simulink model "LCC_C"  (R2026b)
settings: Solver=ode23t  StopTime=5e-6
InitFcn:
  | % LCC-C WPT Inverse Design
  | % All values use SI units
  | 
  | %% 1. Known parameters
  | F = 13.56e6;       % Frequency (Hz)
  | V = 173.2;            % Peak voltage (V), P_in = 500w
  | 
  | L_1 = 486e-9;      % Transmitter coil (H)
  | L_2 = 486e-9; % Receiver coil (H)
  | L21 = 90e-9
  | 
  | R_l = 12.5;        % Load resistance (Ohm)
  | Z_in = 30;         % Target input impedance (Ohm)
  | 
  | Q_1 = 951.1;       % Transmitter quality factor
  | Q_2 = 931;         % Receiver quality factor
  | 
  | %% 2. Derived parameters
  | omega = 2*pi*F;
  | T = 1/F;
  | 
  | % Load quality factor
  | Q_load = omega*L_2/R_l;
  | 
  | % Coupling coefficient from optimal load condition
  | k = sqrt(((Q_2/Q_load)^2-1)/(Q_1*Q_2));
  | 
  | % Mutual inductance
  | M = k*sqrt(L_1*L_2);
  | 
  | % LCC compensation inductor
  | L = M*sqrt(Z_in/R_l);
  | 
  | % LCC parallel compensation capacitor
  | C = 1/(omega^2*L);
  | 
  | % Transmitter series capacitor
  | C_1 = 1/(omega^2*(L_1-L));
  | 
  | % Receiver series capacitor
  | C_2 = 1/(omega^2*(L_2+L21));
  | 
  | %% 3. Additional calculated quantities
  | R_1 = omega*L_1/Q_1;
  | R_2 = omega*L_2/Q_2;
  | 
  | Q_load_opt = Q_2/sqrt(1+k^2*Q_1*Q_2);
  | Z_in_check = (L/M)^2*R_l;
  | 
  | I_in_pk_ideal = V/Z_in;
  | P_in_ideal = V^2/(2*Z_in);
libraries: fl_lib x54, nesl_utility x33
settings Model: Creator=charl  LastModifiedBy=charl
settings SimscapeCC: SimscapeLogType=all  SimscapeNominalValues="[{\"value\":\"1\",\"unit\":\"A\"},{\"value\":\"1\",\"unit\":\"bar\"},{\"value\":\"1\",\"unit\":\"cm^2\"},{\"value\":\"1\",\"unit\":\"cm^3/s\"},{\"value\":\"1\",\"unit\":\"kJ/kg\"},{\"value\":\"1\",\"unit\":\"kW\"},{\"value\":\"1\",\"unit\":\"l\"},{\"value\":\"1\",\"unit\":\"N\"},{\"value\":\"1\",\"unit\":\"N*m\"},{\"value\":\"1\",\"unit\":\"V\"},{\"value\":\"0.001\",\"unit\":\"Wb\"}]"  SimscapeUseEnergyAccounting=off

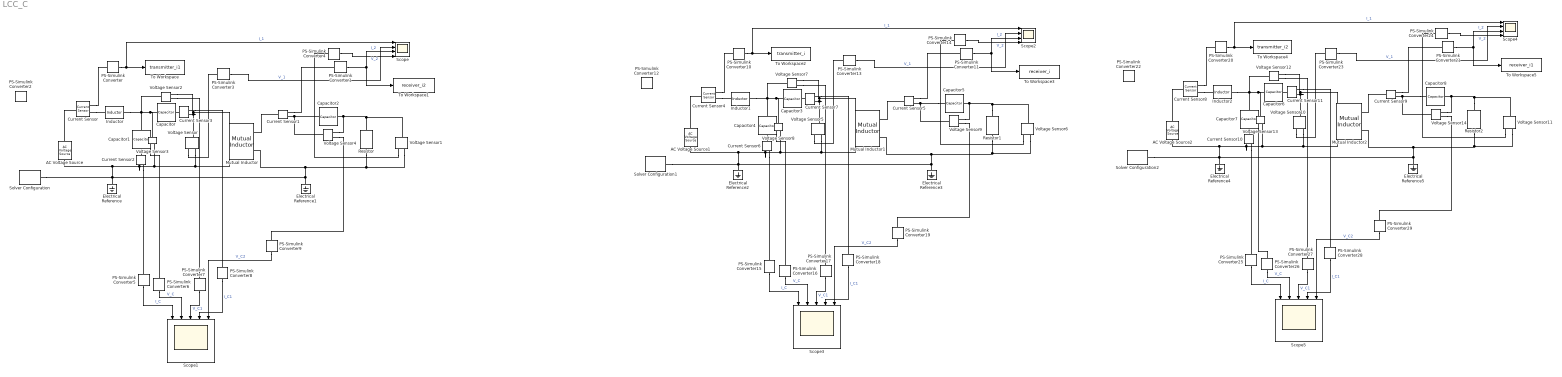
== system LCC_C ==
  AC Voltage Source : fl_lib/Electrical/Electrical Sources/AC Voltage Source  amp=V V  shift=0 deg  frequency=F Hz
  AC Voltage Source1 : fl_lib/Electrical/Electrical Sources/AC Voltage Source  amp=V V  shift=0 deg  frequency=F Hz
  AC Voltage Source2 : fl_lib/Electrical/Electrical Sources/AC Voltage Source  amp=V V  shift=0 deg  frequency=F Hz
  Capacitor : fl_lib/Electrical/Electrical Elements/Capacitor  c=C_1 F  r=1e-6 Ohm  g=0 1/Ohm  i_specify=off  i_priority=None  i=0 A  i_nominal_specify=off  i_nominal_value=1  i_nominal_unit=A  v_specify=off  v_priority=None  v=0 V  v_nominal_specify=off  v_nominal_value=1  v_nominal_unit=V  vc_specify=off  vc_priority=High  vc=0 V  vc_nominal_specify=off  vc_nominal_value=1  vc_nominal_unit=V
  Capacitor1 : fl_lib/Electrical/Electrical Elements/Capacitor  c=C F  r=1e-6 Ohm  g=0 1/Ohm  i_specify=off  i_priority=None  i=0 A  i_nominal_specify=off  i_nominal_value=1  i_nominal_unit=A  v_specify=off  v_priority=None  v=0 V  v_nominal_specify=off  v_nominal_value=1  v_nominal_unit=V  vc_specify=off  vc_priority=High  vc=0 V  vc_nominal_specify=off  vc_nominal_value=1  vc_nominal_unit=V
  Capacitor2 : fl_lib/Electrical/Electrical Elements/Capacitor  c=C_2 F  r=1e-6 Ohm  g=0 1/Ohm  i_specify=off  i_priority=None  i=0 A  i_nominal_specify=off  i_nominal_value=1  i_nominal_unit=A  v_specify=off  v_priority=None  v=0 V  v_nominal_specify=off  v_nominal_value=1  v_nominal_unit=V  vc_specify=off  vc_priority=High  vc=0 V  vc_nominal_specify=off  vc_nominal_value=1  vc_nominal_unit=V
  Capacitor3 : fl_lib/Electrical/Electrical Elements/Capacitor  c=C_1 F  r=1e-6 Ohm  g=0 1/Ohm  i_specify=off  i_priority=None  i=0 A  i_nominal_specify=off  i_nominal_value=1  i_nominal_unit=A  v_specify=off  v_priority=None  v=0 V  v_nominal_specify=off  v_nominal_value=1  v_nominal_unit=V  vc_specify=off  vc_priority=High  vc=0 V  vc_nominal_specify=off  vc_nominal_value=1  vc_nominal_unit=V
  Capacitor4 : fl_lib/Electrical/Electrical Elements/Capacitor  c=C F  r=1e-6 Ohm  g=0 1/Ohm  i_specify=off  i_priority=None  i=0 A  i_nominal_specify=off  i_nominal_value=1  i_nominal_unit=A  v_specify=off  v_priority=None  v=0 V  v_nominal_specify=off  v_nominal_value=1  v_nominal_unit=V  vc_specify=off  vc_priority=High  vc=0 V  vc_nominal_specify=off  vc_nominal_value=1  vc_nominal_unit=V
  Capacitor5 : fl_lib/Electrical/Electrical Elements/Capacitor  c=C_2 F  r=1e-6 Ohm  g=0 1/Ohm  i_specify=off  i_priority=None  i=0 A  i_nominal_specify=off  i_nominal_value=1  i_nominal_unit=A  v_specify=off  v_priority=None  v=0 V  v_nominal_specify=off  v_nominal_value=1  v_nominal_unit=V  vc_specify=off  vc_priority=High  vc=0 V  vc_nominal_specify=off  vc_nominal_value=1  vc_nominal_unit=V
  Capacitor6 : fl_lib/Electrical/Electrical Elements/Capacitor  c=C_1 F  r=1e-6 Ohm  g=0 1/Ohm  i_specify=off  i_priority=None  i=0 A  i_nominal_specify=off  i_nominal_value=1  i_nominal_unit=A  v_specify=off  v_priority=None  v=0 V  v_nominal_specify=off  v_nominal_value=1  v_nominal_unit=V  vc_specify=off  vc_priority=High  vc=0 V  vc_nominal_specify=off  vc_nominal_value=1  vc_nominal_unit=V
  Capacitor7 : fl_lib/Electrical/Electrical Elements/Capacitor  c=C F  r=1e-6 Ohm  g=0 1/Ohm  i_specify=off  i_priority=None  i=0 A  i_nominal_specify=off  i_nominal_value=1  i_nominal_unit=A  v_specify=off  v_priority=None  v=0 V  v_nominal_specify=off  v_nominal_value=1  v_nominal_unit=V  vc_specify=off  vc_priority=High  vc=0 V  vc_nominal_specify=off  vc_nominal_value=1  vc_nominal_unit=V
  Capacitor8 : fl_lib/Electrical/Electrical Elements/Capacitor  c=C_2 F  r=1e-6 Ohm  g=0 1/Ohm  i_specify=off  i_priority=None  i=0 A  i_nominal_specify=off  i_nominal_value=1  i_nominal_unit=A  v_specify=off  v_priority=None  v=0 V  v_nominal_specify=off  v_nominal_value=1  v_nominal_unit=V  vc_specify=off  vc_priority=High  vc=0 V  vc_nominal_specify=off  vc_nominal_value=1  vc_nominal_unit=V
  Current Sensor{,1..11} (12 alike) : fl_lib/Electrical/Electrical Sensors/Current Sensor
  Electrical Reference{,1..5} (6 alike) : fl_lib/Electrical/Electrical Elements/Electrical Reference
  Inductor : fl_lib/Electrical/Electrical Elements/Inductor  l=L H  r=0 Ohm  g=1e-9 1/Ohm  i_specify=off  i_priority=None  i=0 A  i_nominal_specify=off  i_nominal_value=1  i_nominal_unit=A  v_specify=off  v_priority=None  v=0 V  v_nominal_specify=off  v_nominal_value=1  v_nominal_unit=V  i_L_specify=off  i_L_priority=High  i_L=0 A  i_L_nominal_specify=off  i_L_nominal_value=1  i_L_nominal_unit=A
  Inductor1 : fl_lib/Electrical/Electrical Elements/Inductor  l=L H  r=0 Ohm  g=1e-9 1/Ohm  i_specify=off  i_priority=None  i=0 A  i_nominal_specify=off  i_nominal_value=1  i_nominal_unit=A  v_specify=off  v_priority=None  v=0 V  v_nominal_specify=off  v_nominal_value=1  v_nominal_unit=V  i_L_specify=off  i_L_priority=High  i_L=0 A  i_L_nominal_specify=off  i_L_nominal_value=1  i_L_nominal_unit=A
  Inductor2 : fl_lib/Electrical/Electrical Elements/Inductor  l=L H  r=0 Ohm  g=1e-9 1/Ohm  i_specify=off  i_priority=None  i=0 A  i_nominal_specify=off  i_nominal_value=1  i_nominal_unit=A  v_specify=off  v_priority=None  v=0 V  v_nominal_specify=off  v_nominal_value=1  v_nominal_unit=V  i_L_specify=off  i_L_priority=High  i_L=0 A  i_L_nominal_specify=off  i_L_nominal_value=1  i_L_nominal_unit=A
  Mutual Inductor : fl_lib/Electrical/Electrical Elements/Mutual Inductor  L1=L_1 H  L2=L_2 H  perfectCoupling=false  k=0.9  i1_specify=off  i1_priority=None  i1=0 A  i1_nominal_specify=off  i1_nominal_value=1  i1_nominal_unit=A  i2_specify=off  i2_priority=None  i2=0 A  i2_nominal_specify=off  i2_nominal_value=1  i2_nominal_unit=A  v1_specify=off  v1_priority=None  v1=0 V  v1_nominal_specify=off  v1_nominal_value=1  v1_nominal_unit=V  v2_specify=off  v2_priority=None  v2=0 V  v2_nominal_specify=off  v2_nominal_value=1  v2_nominal_unit=V
  Mutual Inductor1 : fl_lib/Electrical/Electrical Elements/Mutual Inductor  L1=L_1 H  L2=L_2 H  perfectCoupling=false  k=0.9  i1_specify=off  i1_priority=None  i1=0 A  i1_nominal_specify=off  i1_nominal_value=1  i1_nominal_unit=A  i2_specify=off  i2_priority=None  i2=0 A  i2_nominal_specify=off  i2_nominal_value=1  i2_nominal_unit=A  v1_specify=off  v1_priority=None  v1=0 V  v1_nominal_specify=off  v1_nominal_value=1  v1_nominal_unit=V  v2_specify=off  v2_priority=None  v2=0 V  v2_nominal_specify=off  v2_nominal_value=1  v2_nominal_unit=V
  Mutual Inductor2 : fl_lib/Electrical/Electrical Elements/Mutual Inductor  L1=L_1 H  L2=L_2 H  perfectCoupling=false  k=0.9  i1_specify=off  i1_priority=None  i1=0 A  i1_nominal_specify=off  i1_nominal_value=1  i1_nominal_unit=A  i2_specify=off  i2_priority=None  i2=0 A  i2_nominal_specify=off  i2_nominal_value=1  i2_nominal_unit=A  v1_specify=off  v1_priority=None  v1=0 V  v1_nominal_specify=off  v1_nominal_value=1  v1_nominal_unit=V  v2_specify=off  v2_priority=None  v2=0 V  v2_nominal_specify=off  v2_nominal_value=1  v2_nominal_unit=V
  PS-Simulink Converter{,1,5,8,10..11,15,18,20..21,25,28} (12 alike) : nesl_utility/PS-Simulink Converter  PhysicalDomain=network_engine_domain  SubClassName=ps_output  LeftPortType=input  RightPortType=output  PseudoPeriodic=off  Frequencies=[]  VectorFormat=inherit  Unit=A  AffineConversion=off
  PS-Simulink Converter12 : nesl_utility/PS-Simulink Converter  PhysicalDomain=network_engine_domain  SubClassName=ps_output  LeftPortType=input  RightPortType=output  PseudoPeriodic=off  Frequencies=[]  VectorFormat=inherit  Unit=inherit  AffineConversion=off
  PS-Simulink Converter{3..4,6..7,9,13..14,16..17,19,23..24,26..27,29} (15 alike) : nesl_utility/PS-Simulink Converter  PhysicalDomain=network_engine_domain  SubClassName=ps_output  LeftPortType=input  RightPortType=output  PseudoPeriodic=off  Frequencies=[]  VectorFormat=inherit  Unit=V  AffineConversion=off
  PS-Simulink Converter2 : nesl_utility/PS-Simulink Converter  PhysicalDomain=network_engine_domain  SubClassName=ps_output  LeftPortType=input  RightPortType=output  PseudoPeriodic=off  Frequencies=[]  VectorFormat=inherit  Unit=inherit  AffineConversion=off
  PS-Simulink Converter22 : nesl_utility/PS-Simulink Converter  PhysicalDomain=network_engine_domain  SubClassName=ps_output  LeftPortType=input  RightPortType=output  PseudoPeriodic=off  Frequencies=[]  VectorFormat=inherit  Unit=inherit  AffineConversion=off
  Resistor : fl_lib/Electrical/Electrical Elements/Resistor  R=R_l Ohm  i_specify=off  i_priority=None  i=0 A  i_nominal_specify=off  i_nominal_value=1  i_nominal_unit=A  v_specify=off  v_priority=None  v=0 V  v_nominal_specify=off  v_nominal_value=1  v_nominal_unit=V
  Resistor1 : fl_lib/Electrical/Electrical Elements/Resistor  R=30 Ohm  i_specify=off  i_priority=None  i=0 A  i_nominal_specify=off  i_nominal_value=1  i_nominal_unit=A  v_specify=off  v_priority=None  v=0 V  v_nominal_specify=off  v_nominal_value=1  v_nominal_unit=V
  Resistor2 : fl_lib/Electrical/Electrical Elements/Resistor  R=50 Ohm  i_specify=off  i_priority=None  i=0 A  i_nominal_specify=off  i_nominal_value=1  i_nominal_unit=A  v_specify=off  v_priority=None  v=0 V  v_nominal_specify=off  v_nominal_value=1  v_nominal_unit=V
  Scope : Scope  NumInputPorts=4
      settings: ActiveDisplayYMinimum=-66.230236522243871  ActiveDisplayYMaximum=66.610915035747723
  Scope1 : Scope  NumInputPorts=5
      settings: ActiveDisplayYMinimum=-66.453081033612648  ActiveDisplayYMaximum=66.8824071595852
  Scope2 : Scope  NumInputPorts=4
      settings: ActiveDisplayYMinimum=-66.230236522243871  ActiveDisplayYMaximum=66.610915035747723  DataLoggingVariableName=ScopeData2
  Scope3 : Scope  NumInputPorts=5
      settings: ActiveDisplayYMinimum=-66.453081033612648  ActiveDisplayYMaximum=66.8824071595852  DataLoggingVariableName=ScopeData3
  Scope4 : Scope  NumInputPorts=4
      settings: ActiveDisplayYMinimum=-66.230236522243871  ActiveDisplayYMaximum=66.610915035747723  DataLoggingVariableName=ScopeData4
  Scope5 : Scope  NumInputPorts=5
      settings: ActiveDisplayYMinimum=-66.453081033612648  ActiveDisplayYMaximum=66.8824071595852  DataLoggingVariableName=ScopeData5
  Solver Configuration : nesl_utility/Solver Configuration  PhysicalDomain=network_engine_domain  SubClassName=solver  LeftPortType=input  RightPortType=generic  Tones=[]  Harmonics=[]  SimulateNoise=off  Profile=off  UseLocalSampling=off  EnableSwitchedLinearOptims=on  FrequencyDomain=off  UseCCode=off  RelTol=0.001  AbsTol=0.001  MinStep=1e-09  ToWorkspace=off  RevertToSquareIcSolve=off  NumHomotopyIterations=100  PhasorMode=off  PhasorModeNumHarmonics=1  ConsistencySolver=NEWTON_XTOL_AFTER_FTOL  CanonicalOrdering=CANONICAL  OptimizeIntermediates=OPTIMIZED  MulticoreSolverChoice=BACKWARD_EULER  IndexReductionMethod=DerivativeReplacement  DoDC=off  ResidualTolerance=1e-09  ConsistencyTolSource=GLOBAL  ConsistencyAbsTol=0.001  ConsistencyRelTol=0.001  ConsistencyTolFactor=0.001  UseLocalSolver=off  LocalSolverChoice=NE_BACKWARD_EULER_ADVANCER  ResolveIndetEquations=on  FunctionEvalNumThread=1  LocalSolverSampleTime=0.001  DoFixedCost=off  MaxNonlinIter=3  MaxModeIter=2  ComputeImpulses=off  ImpulseIterations=2  LinearAlgebra=auto  LinearAlgebraNumThread=0  EquationFormulation=NE_TIME_EF  DelaysMemoryBudget=1024  AutomaticFiltering=on  FilteringTimeConstant=0.001  PartitionStorageMethod=AS_NEEDED  PartitionMemoryBudget=1024  PartitionMethod=BALANCED  MultibodyUseLocalSolver=off  MultibodyLocalSolverChoice=ODE1  MultibodyLocalSolverSampleTime=0.001
  Solver Configuration1 : nesl_utility/Solver Configuration  PhysicalDomain=network_engine_domain  SubClassName=solver  LeftPortType=input  RightPortType=generic  Tones=[]  Harmonics=[]  SimulateNoise=off  Profile=off  UseLocalSampling=off  EnableSwitchedLinearOptims=on  FrequencyDomain=off  UseCCode=off  RelTol=0.001  AbsTol=0.001  MinStep=1e-09  ToWorkspace=off  RevertToSquareIcSolve=off  NumHomotopyIterations=100  PhasorMode=off  PhasorModeNumHarmonics=1  ConsistencySolver=NEWTON_XTOL_AFTER_FTOL  CanonicalOrdering=CANONICAL  OptimizeIntermediates=OPTIMIZED  MulticoreSolverChoice=BACKWARD_EULER  IndexReductionMethod=DerivativeReplacement  DoDC=off  ResidualTolerance=1e-09  ConsistencyTolSource=GLOBAL  ConsistencyAbsTol=0.001  ConsistencyRelTol=0.001  ConsistencyTolFactor=0.001  UseLocalSolver=off  LocalSolverChoice=NE_BACKWARD_EULER_ADVANCER  ResolveIndetEquations=on  FunctionEvalNumThread=1  LocalSolverSampleTime=0.001  DoFixedCost=off  MaxNonlinIter=3  MaxModeIter=2  ComputeImpulses=off  ImpulseIterations=2  LinearAlgebra=auto  LinearAlgebraNumThread=0  EquationFormulation=NE_TIME_EF  DelaysMemoryBudget=1024  AutomaticFiltering=on  FilteringTimeConstant=0.001  PartitionStorageMethod=AS_NEEDED  PartitionMemoryBudget=1024  PartitionMethod=BALANCED  MultibodyUseLocalSolver=off  MultibodyLocalSolverChoice=ODE1  MultibodyLocalSolverSampleTime=0.001
  Solver Configuration2 : nesl_utility/Solver Configuration  PhysicalDomain=network_engine_domain  SubClassName=solver  LeftPortType=input  RightPortType=generic  Tones=[]  Harmonics=[]  SimulateNoise=off  Profile=off  UseLocalSampling=off  EnableSwitchedLinearOptims=on  FrequencyDomain=off  UseCCode=off  RelTol=0.001  AbsTol=0.001  MinStep=1e-09  ToWorkspace=off  RevertToSquareIcSolve=off  NumHomotopyIterations=100  PhasorMode=off  PhasorModeNumHarmonics=1  ConsistencySolver=NEWTON_XTOL_AFTER_FTOL  CanonicalOrdering=CANONICAL  OptimizeIntermediates=OPTIMIZED  MulticoreSolverChoice=BACKWARD_EULER  IndexReductionMethod=DerivativeReplacement  DoDC=off  ResidualTolerance=1e-09  ConsistencyTolSource=GLOBAL  ConsistencyAbsTol=0.001  ConsistencyRelTol=0.001  ConsistencyTolFactor=0.001  UseLocalSolver=off  LocalSolverChoice=NE_BACKWARD_EULER_ADVANCER  ResolveIndetEquations=on  FunctionEvalNumThread=1  LocalSolverSampleTime=0.001  DoFixedCost=off  MaxNonlinIter=3  MaxModeIter=2  ComputeImpulses=off  ImpulseIterations=2  LinearAlgebra=auto  LinearAlgebraNumThread=0  EquationFormulation=NE_TIME_EF  DelaysMemoryBudget=1024  AutomaticFiltering=on  FilteringTimeConstant=0.001  PartitionStorageMethod=AS_NEEDED  PartitionMemoryBudget=1024  PartitionMethod=BALANCED  MultibodyUseLocalSolver=off  MultibodyLocalSolverChoice=ODE1  MultibodyLocalSolverSampleTime=0.001
  To Workspace : ToWorkspace  VariableName=transmitter_i1  SaveFormat=Timeseries  SampleTime=-1
  To Workspace1 : ToWorkspace  VariableName=receiver_i2  SaveFormat=Timeseries  SampleTime=-1
  To Workspace2 : ToWorkspace  VariableName=transmitter_i  SaveFormat=Timeseries  SampleTime=-1
  To Workspace3 : ToWorkspace  VariableName=receiver_i  SaveFormat=Timeseries  SampleTime=-1
  To Workspace4 : ToWorkspace  VariableName=transmitter_i2  SaveFormat=Timeseries  SampleTime=-1
  To Workspace5 : ToWorkspace  VariableName=receiver_i1  SaveFormat=Timeseries  SampleTime=-1
  Voltage Sensor{,1..14} (15 alike) : fl_lib/Electrical/Electrical Sensors/Voltage Sensor
  wires:
  PS-Simulink Converter/1 -> Scope/1, To Workspace/1  "I_1"
  PS-Simulink Converter1/1 -> Scope/3, To Workspace1/1  "I_2"
  PS-Simulink Converter4/1 -> Scope/4  "V_2"
  PS-Simulink Converter3/1 -> Scope/2  "V_1"
  PS-Simulink Converter5/1 -> Scope1/1  "I_C"
  PS-Simulink Converter6/1 -> Scope1/2  "V_C"
  PS-Simulink Converter7/1 -> Scope1/3  "V_C1"
  PS-Simulink Converter8/1 -> Scope1/4  "I_C1"
  PS-Simulink Converter9/1 -> Scope1/5  "V_C2"
  PS-Simulink Converter10/1 -> Scope2/1, To Workspace2/1  "I_1"
  PS-Simulink Converter15/1 -> Scope3/1  "I_C"
  PS-Simulink Converter19/1 -> Scope3/5  "V_C2"
  PS-Simulink Converter11/1 -> Scope2/3, To Workspace3/1  "I_2"
  PS-Simulink Converter16/1 -> Scope3/2  "V_C"
  PS-Simulink Converter13/1 -> Scope2/2  "V_1"
  PS-Simulink Converter17/1 -> Scope3/3  "V_C1"
  PS-Simulink Converter18/1 -> Scope3/4  "I_C1"
  PS-Simulink Converter14/1 -> Scope2/4  "V_2"
  PS-Simulink Converter20/1 -> Scope4/1, To Workspace4/1  "I_1"
  PS-Simulink Converter25/1 -> Scope5/1  "I_C"
  PS-Simulink Converter29/1 -> Scope5/5  "V_C2"
  PS-Simulink Converter21/1 -> Scope4/3, To Workspace5/1  "I_2"
  PS-Simulink Converter26/1 -> Scope5/2  "V_C"
  PS-Simulink Converter23/1 -> Scope4/2  "V_1"
  PS-Simulink Converter27/1 -> Scope5/3  "V_C1"
  PS-Simulink Converter28/1 -> Scope5/4  "I_C1"
  PS-Simulink Converter24/1 -> Scope4/4  "V_2"
  connections:
  Inductor/RConn1 -- Voltage Sensor3/LConn1 -- Capacitor/LConn1 -- Capacitor1/LConn1 -- Voltage Sensor2/LConn1
  Current Sensor/LConn1 -- AC Voltage Source/LConn1
  Current Sensor/RConn2 -- Inductor/LConn1
  Current Sensor/RConn1 -- PS-Simulink Converter/LConn1
  Current Sensor1/RConn1 -- PS-Simulink Converter1/LConn1
  Current Sensor1/LConn1 -- Mutual Inductor/RConn1
  Voltage Sensor/LConn1 -- Voltage Sensor2/RConn2 -- Mutual Inductor/LConn1 -- Current Sensor3/RConn2
  Capacitor2/RConn1 -- Voltage Sensor4/RConn2 -- Voltage Sensor1/LConn1 -- Resistor/LConn1
  Current Sensor1/RConn2 -- Voltage Sensor4/LConn1 -- Capacitor2/LConn1
  Voltage Sensor3/RConn2 -- Voltage Sensor/RConn2 -- Mutual Inductor/LConn2 -- Current Sensor2/RConn2 -- AC Voltage Source/RConn1 -- Solver Configuration/RConn1 -- Voltage Sensor1/RConn2 -- Resistor/RConn1 -- Mutual Inductor/RConn2 -- Electrical Reference1/LConn1 -- Electrical Reference/LConn1
  Voltage Sensor/RConn1 -- PS-Simulink Converter3/LConn1
  Voltage Sensor1/RConn1 -- PS-Simulink Converter4/LConn1
  Current Sensor2/LConn1 -- Capacitor1/RConn1
  Current Sensor3/LConn1 -- Capacitor/RConn1
  Current Sensor2/RConn1 -- PS-Simulink Converter5/LConn1
  Voltage Sensor3/RConn1 -- PS-Simulink Converter6/LConn1
  Voltage Sensor2/RConn1 -- PS-Simulink Converter7/LConn1
  Current Sensor3/RConn1 -- PS-Simulink Converter8/LConn1
  Voltage Sensor4/RConn1 -- PS-Simulink Converter9/LConn1
  Resistor1/LConn1 -- Capacitor5/RConn1 -- Voltage Sensor9/RConn2 -- Voltage Sensor6/LConn1
  Current Sensor7/RConn2 -- Voltage Sensor5/LConn1 -- Voltage Sensor7/RConn2 -- Mutual Inductor1/LConn1
  Mutual Inductor1/RConn2 -- Voltage Sensor8/RConn2 -- Voltage Sensor5/RConn2 -- Mutual Inductor1/LConn2 -- Current Sensor6/RConn2 -- AC Voltage Source1/RConn1 -- Solver Configuration1/RConn1 -- Electrical Reference2/LConn1 -- Electrical Reference3/LConn1 -- Voltage Sensor6/RConn2 -- Resistor1/RConn1
  Capacitor5/LConn1 -- Current Sensor5/RConn2 -- Voltage Sensor9/LConn1
  Capacitor3/LConn1 -- Inductor1/RConn1 -- Capacitor4/LConn1 -- Voltage Sensor7/LConn1 -- Voltage Sensor8/LConn1
  Current Sensor6/RConn1 -- PS-Simulink Converter15/LConn1
  Voltage Sensor9/RConn1 -- PS-Simulink Converter19/LConn1
  Current Sensor4/RConn1 -- PS-Simulink Converter10/LConn1
  Current Sensor5/LConn1 -- Mutual Inductor1/RConn1
  Voltage Sensor7/RConn1 -- PS-Simulink Converter17/LConn1
  Current Sensor7/LConn1 -- Capacitor3/RConn1
  Voltage Sensor5/RConn1 -- PS-Simulink Converter13/LConn1
  Current Sensor6/LConn1 -- Capacitor4/RConn1
  Voltage Sensor6/RConn1 -- PS-Simulink Converter14/LConn1
  Current Sensor7/RConn1 -- PS-Simulink Converter18/LConn1
  Current Sensor4/LConn1 -- AC Voltage Source1/LConn1
  Voltage Sensor8/RConn1 -- PS-Simulink Converter16/LConn1
  Current Sensor4/RConn2 -- Inductor1/LConn1
  Current Sensor5/RConn1 -- PS-Simulink Converter11/LConn1
  Resistor2/LConn1 -- Capacitor8/RConn1 -- Voltage Sensor14/RConn2 -- Voltage Sensor11/LConn1
  Current Sensor11/RConn2 -- Voltage Sensor10/LConn1 -- Voltage Sensor12/RConn2 -- Mutual Inductor2/LConn1
  Mutual Inductor2/RConn2 -- Voltage Sensor13/RConn2 -- Voltage Sensor10/RConn2 -- Mutual Inductor2/LConn2 -- Current Sensor10/RConn2 -- AC Voltage Source2/RConn1 -- Solver Configuration2/RConn1 -- Electrical Reference4/LConn1 -- Electrical Reference5/LConn1 -- Voltage Sensor11/RConn2 -- Resistor2/RConn1
  Capacitor8/LConn1 -- Current Sensor9/RConn2 -- Voltage Sensor14/LConn1
  Capacitor6/LConn1 -- Inductor2/RConn1 -- Capacitor7/LConn1 -- Voltage Sensor12/LConn1 -- Voltage Sensor13/LConn1
  Current Sensor10/RConn1 -- PS-Simulink Converter25/LConn1
  Voltage Sensor14/RConn1 -- PS-Simulink Converter29/LConn1
  Current Sensor8/RConn1 -- PS-Simulink Converter20/LConn1
  Current Sensor9/LConn1 -- Mutual Inductor2/RConn1
  Voltage Sensor12/RConn1 -- PS-Simulink Converter27/LConn1
  Current Sensor11/LConn1 -- Capacitor6/RConn1
  Voltage Sensor10/RConn1 -- PS-Simulink Converter23/LConn1
  Current Sensor10/LConn1 -- Capacitor7/RConn1
  Voltage Sensor11/RConn1 -- PS-Simulink Converter24/LConn1
  Current Sensor11/RConn1 -- PS-Simulink Converter28/LConn1
  Current Sensor8/LConn1 -- AC Voltage Source2/LConn1
  Voltage Sensor13/RConn1 -- PS-Simulink Converter26/LConn1
  Current Sensor8/RConn2 -- Inductor2/LConn1
  Current Sensor9/RConn1 -- PS-Simulink Converter21/LConn1
